simulink subsystem "PieroControladoPosZ"  (R2022b)
settings: Solver=VariableStepAuto  StartTime=0.0  StopTime=10.0  RelTol=1e-3
undefined symbols (not defined in the file or in its folder): DiscIntNeverNeededParam
settings Model: Creator=miriamfreiriasanjuan  LastModifiedBy=miriamfreiriasanjuan

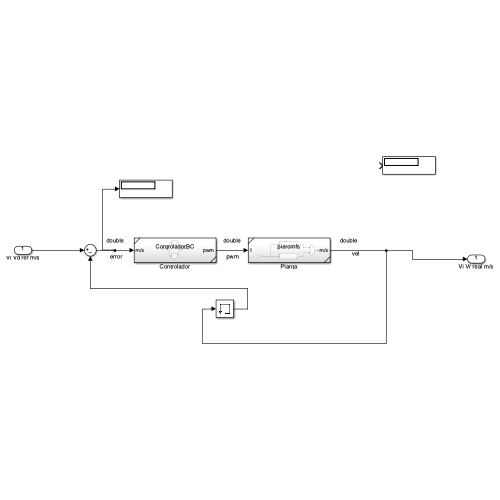
[thumbnail: Simulink's stored preview of the top-level diagram]
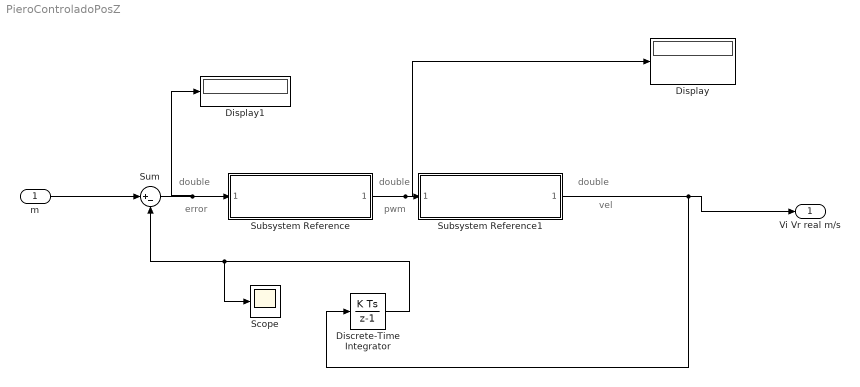
== system PieroControladoPosZ ==
  note: pwm
  note: double
  note: double
  note: error
  note: double
  note: vel
  m : Inport  OutDataTypeStr=double  PortDimensions=2
  Discrete-Time Integrator : DiscreteIntegrator  SampleTime=-1  ICPrevOutput=DiscIntNeverNeededParam  ICPrevScaledInput=DiscIntNeverNeededParam
  Display : Display
  Display1 : Display
  Scope : Scope
  Subsystem Reference : Subsystem  ReferencedSubsystem=ControladorPos1mZ
  Subsystem Reference1 : Subsystem  ReferencedSubsystem=pieromfsZ
  Sum : Sum  Inputs=|+-
  Vi Vr real m/s : Outport
  wires:
  m/1 -> Sum/1
  Sum/1 -> Display1/1, Subsystem Reference/1
  Subsystem Reference/1 -> Subsystem Reference1/1, Display/1
  Discrete-Time Integrator/1 -> Sum/2, Scope/1
  Subsystem Reference1/1 -> Vi Vr real m/s/1, Discrete-Time Integrator/1
